simulink library "sm_car_scene_track_mallory_park_obstacle"  (R2025a)
settings: Solver=VariableStepAuto  StartTime=0.0  StopTime=10.0  RelTol=1e-3
undefined symbols (not defined in the file or in its folder): Scene
libraries: simulink x2, Object_Traffic_Light x2, Driver_Override_vx_Obstacle x1, Scene_Utilities x1
Description:
  | Scene of Simscape Vehicle Templates Library
  | 
  | Copyright 2018-2026 The MathWorks, Inc.
settings Model: Creator=smiller  LastModifiedBy=smiller
settings SolverCC: AlgebraicLoopSolver=TrustRegion
settings DataIOCC: ReturnWorkspaceOutputs=off
settings OptimizationCC: ReuseModelBlockBuffer=off
settings DebuggingCC: UnconnectedInputMsg=warning  UnconnectedOutputMsg=warning  UnconnectedLineMsg=warning  ArithmeticOperatorsInVariantConditions=warning
settings ModelReferenceCC: EnableRefExpFcnMdlSchedulingChecks=on
settings SFSimCC: CustomCodeUndefinedFunction=UseInterfaceOnly
settings RTWCC: GPUComputeCapability=3.5  DLArmComputeVersion=19.05

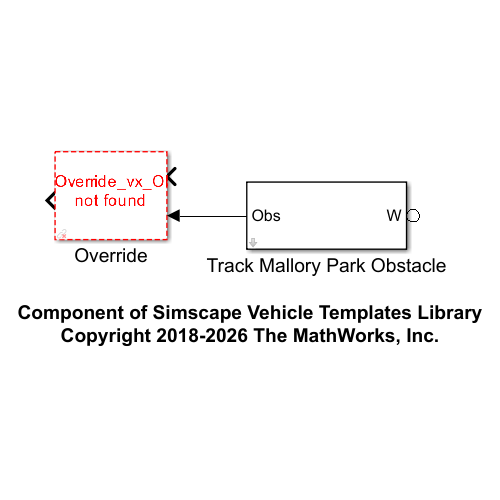
[thumbnail: Simulink's stored preview of the top-level diagram]
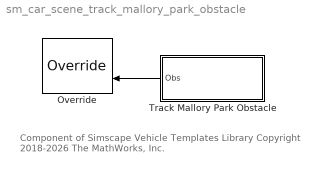
== system sm_car_scene_track_mallory_park_obstacle ==
  note: Component of Simscape Vehicle Templates Library
      | Copyright 2018-2026 The MathWorks, Inc.
  Override : Driver_Override_vx_Obstacle/Override  override=Scene.Mallory_Park_Obstacle.Override
  Track Mallory Park Obstacle : Subsystem  mask{scene_data=Scene.Mallory_Park_Obstacle}
      mask prompts: scene_data "Data (structure)"
  wires:
  Track Mallory Park Obstacle/1(Obs) -> Override/2

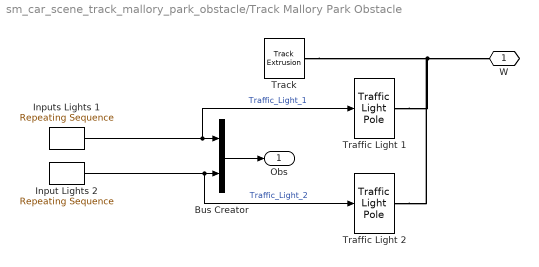
== system sm_car_scene_track_mallory_park_obstacle/Track Mallory Park Obstacle ==
  Bus Creator : BusCreator  Inputs=2
  Input Lights 2 : simulink/Sources/Repeating Sequence  rep_seq_t=scene_data.Traffic_Light_2.lamp.t  rep_seq_y=scene_data.Traffic_Light_2.lamp.RYG
  Inputs Lights 1 : simulink/Sources/Repeating Sequence  rep_seq_t=scene_data.Traffic_Light_1.lamp.t  rep_seq_y=scene_data.Traffic_Light_1.lamp.RYG
  Track : Scene_Utilities/Track Extrusion  track_ctrline=scene_data.Track.ctrline  track_w=scene_data.Track.w  track_h=scene_data.Track.h  track_x=scene_data.Track.x  track_y=scene_data.Track.y  track_z=scene_data.Track.z  track_yaw=scene_data.Track.yaw  track_clr=scene_data.Track.clr  track_opc=scene_data.Track.opc
  Traffic Light 1 : Object_Traffic_Light/Traffic Light Pole  clr_tlp_housing=scene_data.Traffic_Light_1.clr  offset_tlp=[scene_data.Traffic_Light_1.x scene_data.Traffic_Light_1.y scene_data.Traffic_Light_1.z]  orient_tlp=scene_data.Traffic_Light_1.yaw  pole_height_tlp=scene_data.Traffic_Light_1.pole_h
  Traffic Light 2 : Object_Traffic_Light/Traffic Light Pole  clr_tlp_housing=scene_data.Traffic_Light_2.clr  offset_tlp=[scene_data.Traffic_Light_2.x scene_data.Traffic_Light_2.y scene_data.Traffic_Light_2.z]  orient_tlp=scene_data.Traffic_Light_2.yaw  pole_height_tlp=scene_data.Traffic_Light_2.pole_h
  W : PMIOPort  Side=Left
  Obs : Outport  VectorParamsAs1DForOutWhenUnconnected=off
  wires:
  Inputs Lights 1/1 -> Traffic Light 1/1, Bus Creator/1  "Traffic_Light_1"
  Bus Creator/1 -> Obs/1
  Input Lights 2/1 -> Traffic Light 2/1, Bus Creator/2  "Traffic_Light_2"
  connections:
  Track/RConn1 -- Traffic Light 2/RConn1 -- Traffic Light 1/RConn1 -- W/RConn1
